simulink model "task61_closed_loop_model"  (R2024b)
settings: Solver=ode4  StartTime=0.0  StopTime=5  FixedStep=0.001  RelTol=1e-3
undefined symbols (not defined in the file or in its folder): task61_Ki, task61_Kp, task61_plant_den, task61_plant_num, task61_reference_rad_s, task61_step_time_s, task61_voltage_limit_V
settings Model: Creator=yanya  LastModifiedBy=yanya

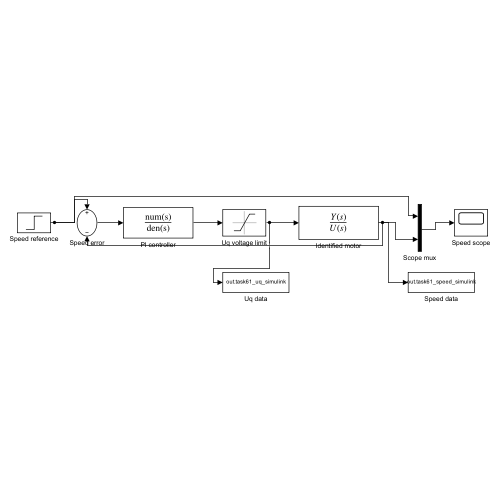
[thumbnail: Simulink's stored preview of the top-level diagram]
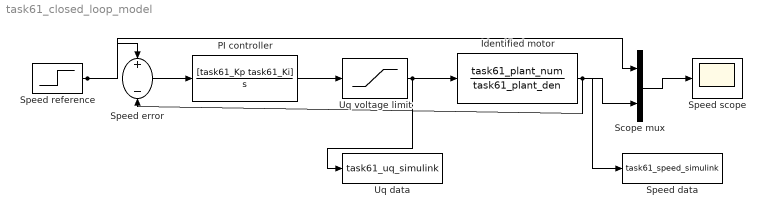
== system task61_closed_loop_model ==
  Identified motor : TransferFcn  Numerator=task61_plant_num  Denominator=task61_plant_den
  PI controller : TransferFcn  Numerator=[task61_Kp task61_Ki]  Denominator=[1 0]
  Scope mux : Mux  Inputs=2
  Speed data : ToWorkspace  VariableName=task61_speed_simulink  SaveFormat=Structure With Time  SampleTime=-1
  Speed error : Sum  Inputs=+-
  Speed reference : Step  Time=task61_step_time_s  After=task61_reference_rad_s  SampleTime=0
  Speed scope : Scope
  Uq data : ToWorkspace  VariableName=task61_uq_simulink  SaveFormat=Structure With Time  SampleTime=-1
  Uq voltage limit : Saturate  UpperLimit=task61_voltage_limit_V  LowerLimit=-task61_voltage_limit_V
  wires:
  Speed reference/1 -> Speed error/1, Scope mux/1
  Speed error/1 -> PI controller/1
  PI controller/1 -> Uq voltage limit/1
  Uq voltage limit/1 -> Identified motor/1, Uq data/1
  Identified motor/1 -> Speed error/2, Scope mux/2, Speed data/1
  Scope mux/1 -> Speed scope/1
